simulink model "FSI10"  (R2024b)
settings: Solver=FixedStepAuto  StartTime=0.0  StopTime=t_stop  FixedStep=Ts  RelTol=1e-3
values from neighbouring files (symbols this model uses):
  c = 1    [FSI10WS.m]
  I = out.EX3.signals.values    [FSI03WS.m]    (also in FSI05WS.m = out.ScopeData.signals(2).values; FSI06WS.m = out.ScopeData1.signals(2).values; FSI07WS.m = out.ScopeData3.signals(2).values; FSI10WS.m = 0.096)
  k = 50000    [FSI04WS.m]    (also in FSI08WS.m = 986.960440109; FSI09WS.m = 15791.3670417; FSI10WS.m = 1480)
  M = 0    [FSI05WS.m]    (also in FSI06WS.m = 0.2; FSI07WS.m = 0.04; FSI10WS.m = 3)
  omega1 = 0    [FSI10WS.m]
  phi1 = 0    [FSI10WS.m]
  swich = -1    [FSI08WS.m]    (also in FSI09WS.m; FSI10WS.m)
settings Model: Creator=fmiro  LastModifiedBy=fmiro

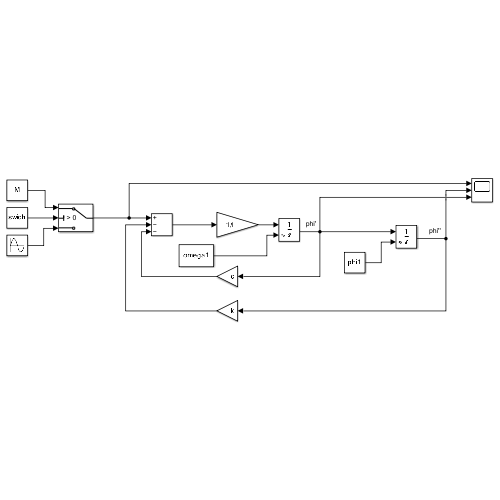
[thumbnail: Simulink's stored preview of the top-level diagram]
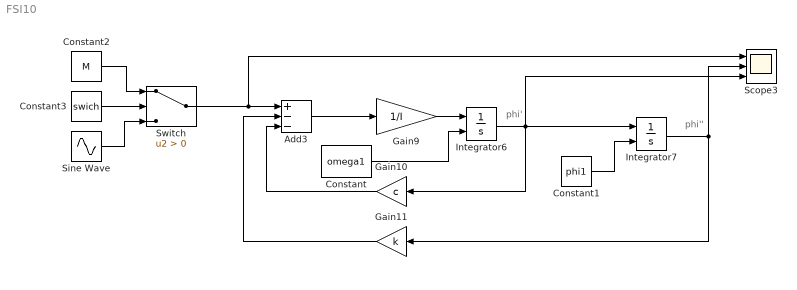
== system FSI10 ==
  note: phi''
  note: phi'
  Add3 : Sum  Inputs=+--
  Constant : Constant  Value=omega1
  Constant1 : Constant  Value=phi1
  Constant2 : Constant  Value=M
  Constant3 : Constant  Value=swich
  Gain10 : Gain  Gain=c
  Gain11 : Gain  Gain=k
  Gain9 : Gain  Gain=1/I
  Integrator6 : Integrator  InitialConditionSource=external
  Integrator7 : Integrator  InitialConditionSource=external
  Scope3 : Scope  NumInputPorts=3
  Sine Wave : Sin  Amplitude=3  Frequency=100  SampleTime=0
  Switch : Switch  Criteria=u2 > Threshold  SaturateOnIntegerOverflow=off  InputSameDT=off
  wires:
  Gain9/1 -> Integrator6/1
  Gain11/1 -> Add3/2
  Integrator6/1 -> Scope3/3, Integrator7/1, Gain10/1
  Add3/1 -> Gain9/1
  Integrator7/1 -> Scope3/2, Gain11/1
  Gain10/1 -> Add3/3
  Constant/1 -> Integrator6/2
  Constant1/1 -> Integrator7/2
  Switch/1 -> Scope3/1, Add3/1
  Constant2/1 -> Switch/1
  Sine Wave/1 -> Switch/3
  Constant3/1 -> Switch/2
